simulink model "OpenLoopDrive"  (R2026b)
settings: Solver=VariableStepAuto
undefined symbols (not defined in the file or in its folder): open_loop_drive_parameters
settings Model: Creator=24322  LastModifiedBy=24322

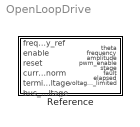
== system OpenLoopDrive ==
  Reference : Subsystem  mask{openLoopCfg=open_loop_drive_parameters()}
      mask prompts: openLoopCfg "Software field and interlock configuration"

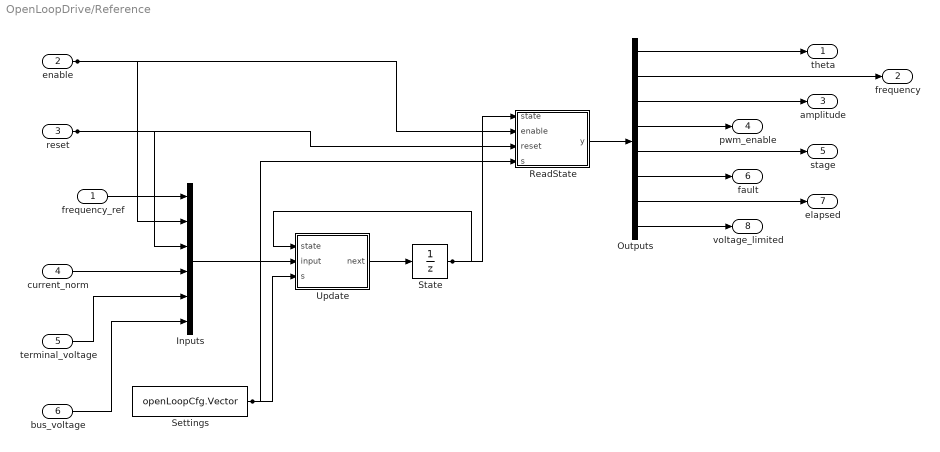
== system OpenLoopDrive/Reference ==
  frequency_ref : Inport  SampleTime=openLoopCfg.Ts
  enable : Inport  Port=2  SampleTime=openLoopCfg.Ts
  reset : Inport  Port=3  SampleTime=openLoopCfg.Ts
  current_norm : Inport  Port=4  SampleTime=openLoopCfg.Ts
  terminal_voltage : Inport  Port=5  SampleTime=openLoopCfg.Ts
  bus_voltage : Inport  Port=6  SampleTime=openLoopCfg.Ts
  Inputs : Mux  Inputs=6
  Outputs : Demux  Outputs=8
  ReadState : MATLAB Function  TreatAsAtomicUnit=on
  Settings : Constant  Value=openLoopCfg.Vector
  State : UnitDelay  InitialCondition=openLoopCfg.State0  SampleTime=openLoopCfg.Ts
  Update : MATLAB Function  TreatAsAtomicUnit=on
  theta : Outport
  frequency : Outport  Port=2
  amplitude : Outport  Port=3
  pwm_enable : Outport  Port=4
  stage : Outport  Port=5
  fault : Outport  Port=6
  elapsed : Outport  Port=7
  voltage_limited : Outport  Port=8
  wires:
  Outputs/8 -> voltage_limited/1
  Outputs/7 -> elapsed/1
  Outputs/6 -> fault/1
  Outputs/5 -> stage/1
  Outputs/4 -> pwm_enable/1
  Outputs/3 -> amplitude/1
  Outputs/2 -> frequency/1
  Outputs/1 -> theta/1
  bus_voltage/1 -> Inputs/6
  terminal_voltage/1 -> Inputs/5
  current_norm/1 -> Inputs/4
  frequency_ref/1 -> Inputs/1
  ReadState/1(y) -> Outputs/1
  reset/1 -> ReadState/3(reset), Inputs/3
  enable/1 -> ReadState/2(enable), Inputs/2
  Update/1(next) -> State/1
  Settings/1 -> Update/3(s), ReadState/4(s)
  Inputs/1 -> Update/2(input)
  State/1 -> ReadState/1(state), Update/1(state)

== matlab function OpenLoopDrive/Reference/ReadState ==
  data: state input; y output; enable input; reset input; s input
function y=open_loop_drive_output(state,enable,reset,s)
%OPEN_LOOP_DRIVE_OUTPUT Held-state output; measured voltage never feeds through.
% y: theta,frequency,amplitude,pwm_enable,stage,fault,elapsed,voltage_limited.
%#codegen
y=[state(3);state(4);state(5);cast(0,'like',state);state(1);state(6);state(2)*s(1);state(8)];
if ~isfinite(enable)||~isfinite(reset)||enable~=1||reset~=0
    y(1)=s(18);y(2:8)=0;return
end
if state(1)==2||state(1)==3,y(4)=1;else,y(2:3)=0;end
end

== matlab function OpenLoopDrive/Reference/Update ==
  data: state input; next output; input input; s input
function next=open_loop_drive_update(state,input,s)
%OPEN_LOOP_DRIVE_UPDATE State-only oscillator; no rotor angle or speed input.
% state: stage,count,theta,frequency,amplitude,fault,low_count,voltage_limited.
% input: electrical_frequency_Hz,enable,reset,current_norm,terminal_voltage,bus.
%#codegen
next=state;s=cast(s,'like',state);u=cast(input,'like',state);
if (isfinite(u(2))&&u(2)==0)||(isfinite(u(3))&&u(3)==1)
    next=zeros(8,1,'like',state);next(3)=s(18);return
end
if ~all(isfinite(u))||u(6)<=0||u(4)<0||u(5)<0|| ...
        (u(2)~=0&&u(2)~=1)||(u(3)~=0&&u(3)~=1)
    next(1)=7;next(6)=2;next(4:5)=0;return
end
if state(1)==7,return;end
if u(4)>s(17),next(1)=7;next(6)=1;next(4:5)=0;return;end
stage=state(1);count=state(2)+1;next(2)=count;next(8)=0;
if stage==0
    next(1)=1;next(2)=0;
elseif stage==1
    low=cast(0,'like',state);
    if u(5)<=s(6)&&u(4)<=s(7),low=state(7)+1;end
    next(7)=low;
    if low>=s(5),next(1)=2;next(2)=0;
    elseif count>=s(8),next(1)=7;next(6)=3;end
elseif stage==2
    next(3)=s(18);next(4)=0;next(5)=s(11)*min(count/s(10),1);
    if count>=s(9),next(1)=3;next(2)=0;end
elseif stage==3
    requested=min(max(u(1),-s(3)),s(3));step=s(4)*s(1);
    next(4)=state(4)+min(max(requested-state(4),-step),step);
    next(3)=atan2(sin(state(3)+2*pi*s(1)*state(4)),cos(state(3)+2*pi*s(1)*state(4)));
    if s(2)==1,amplitude=s(12);
    else
        requestedAmplitude=s(15)+s(14)*abs(next(4));
        amplitude=min(requestedAmplitude,u(6)*s(16));
        next(8)=cast(requestedAmplitude>amplitude,'like',state);
    end
    step=s(13)*s(1);next(5)=state(5)+min(max(amplitude-state(5),-step),step);
else
    next(1)=7;next(6)=4;next(4:5)=0;
end
end
